simulink model "hw_CS1A_seq"  (R2025b)
settings: Solver=FixedStepAuto  StartTime=0.0  StopTime=inf  RelTol=1e-3  EnableMultiTasking=on
InitFcn:
  | run(fullfile(fileparts(get_param(bdroot,'FileName')),'Hardware_settings.m'));
  | run(fullfile(fileparts(get_param(bdroot,'FileName')),'ref_sequence_settings.m'));
StopFcn:
  | run(fullfile(fileparts(get_param(bdroot,'FileName')),'Hardware_data_save.m'));
values from neighbouring files (symbols this model uses):
  ref_hold_s = 8    [ref_sequence_settings.m]
  ref_seq_deg = [45 -45 90 0 -90 0]    [ref_sequence_settings.m]
  ts = 1/1000    (= 0.001)    [Hardware_settings.m]    (also in data_test_06.mat; qube_model.m)
libraries: simulink_extras x4, simulink x3, arduinolib x1
settings Model: SimulationMode=external  ExtModeTrigDuration=2  Creator=ricardoaguilera  LastModifiedBy=jaylen
settings SolverCC: AutoInsertRateTranBlk=on
settings DataIOCC: ReturnWorkspaceOutputs=off
settings OptimizationCC: EnhancedBackFolding=on  PassReuseOutputArgsAs=Individual arguments  ZeroExternalMemoryAtStartup=off  ZeroInternalMemoryAtStartup=off  MaxStackSize=64  OptimizeBlockOrder=speed  DifferentSizesBufferReuse=on  OptimizationCustomize=off  EfficientTunableParamExpr=on
settings DebuggingCC: ParameterTunabilityLossMsg=error
settings HardwareCC: ProdBitPerPointer=32.0  ProdBitPerSizeT=32.0  ProdBitPerPtrDiffT=32.0  ProdLargestAtomicInteger=Long  ProdLargestAtomicFloat=Double  ProdWordSize=32.0  ProdHWDeviceType=ARM Compatible->ARM Cortex
settings SFSimCC: MATLABDynamicMemAlloc=off
settings RTWCC: SystemTargetFile=ert.tlc  HardwareBoard=Teensy 4.1 (Arduino Compatible)  TemplateMakefile=ert_default_tmf  Toolchain=Arduino ARM M7  BuildConfiguration=Faster Runs  Description=Embedded Coder
settings CodeAppCC: ForceParamTrailComments=on  IgnoreCustomStorageClasses=off  OperatorAnnotations=on  SimulinkDataObjDesc=on  SFDataObjDesc=on  InsertBlockDesc=on
settings ERTTargetCC: ExtModeTransport=3.0  ExtModeStaticAlloc=on  ExtModeAutomaticAllocSize=off  ExtModeStaticAllocSize=65536.0  ExtModeMexFile=ext_xcp  ExtModeIntrfLevel=Level2 - Open  InlinedParameterPlacement=Hierarchical  SupportContinuousTime=on  SupportVariableSizeSignals=on

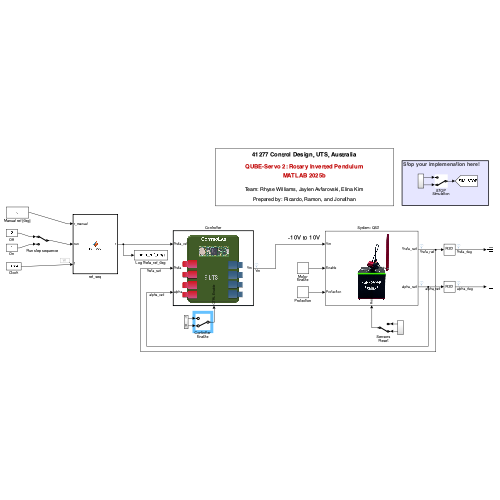
[thumbnail: Simulink's stored preview of the top-level diagram]
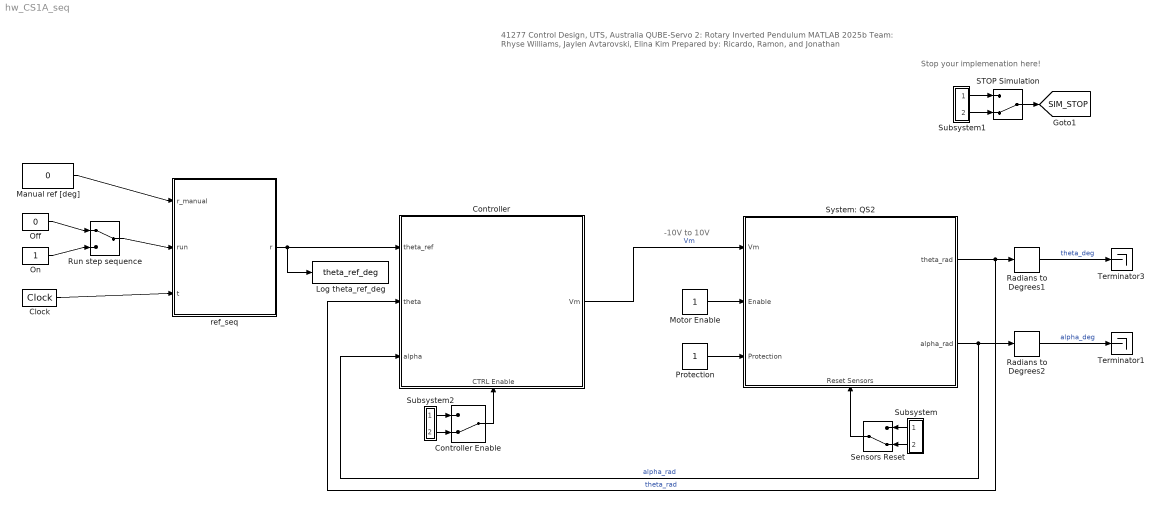
== system hw_CS1A_seq ==
  note: Stop your implemenation here!
  note: -10V to 10V
  note: 41277 Control Design, UTS, Australia
      |
      | QUBE-Servo 2: Rotary Inverted Pendulum
      |
      | MATLAB 2025b
      |
      | Team: Rhyse Williams, Jaylen Avtarovski, Elina Kim
      |
      | Prepared by: Ricardo, Ramon, and Jonathan
  Clock : DigitalClock  SampleTime=ts
  Controller : Subsystem  TreatAsAtomicUnit=on
      settings: PortSchema="{\"entries\":[{\"content\":{\"sides\":[{\"content\":{\"connectorIds\":[\"In1\",\"In2\",\"In3\"]},\"type\":\"ConnectorPlacement.EquallySpacedRectSide\",\"uuid\":\"0746f990-c749-44b4-b231-71e9c63a70c9\"},{\"content\":{\"connectorIds\":[\"Out1\"],\"side\":\"RIGHT\"},\"type\":\"ConnectorPlacement.EquallySpacedRectSide\",\"uuid\":\"2be26398-fce4-47ae-bcef-dcf9a7bb9bcb\"},{\"content\":{\"side\":\"TOP\"},\"type\":\"ConnectorPlacement.EquallySpacedRectSide\",\"uuid\":\"03fd616b-3dd6-472f-b1cd-bcbe330f410d\"},{\"content\":{\"connectorIds\":[\"In4\"],\"side\":\"BOTTOM\"},\"type\":\"ConnectorPlacement.EquallySpacedRectSide\",\"uuid\":\"e0197938-1dca-4730-aea1-41c64defbdb5\"}]},\"type\":\"ConnectorPlacement.EquallySpacedConnector\",\"uuid\":\"8db17840-dba9-44ab-b10b-ffa616c53e04\"}],\"packageUris\":[\"http://schema.mathworks.com/mf0/Connector/R2020b\"],\"version\":\"1.0\"}"
      mask Display: image('Board.png');
  Controller Enable : ManualSwitch  CurrentSetting=0
  Log theta_ref_deg : ToWorkspace  VariableName=theta_ref_deg  SampleTime=-1
  Manual ref [deg] : Constant  Value=0
  Motor Enable : Constant
  Off : Constant  Value=0
  On : Constant
  Protection : Constant
  Radians to Degrees1 : simulink_extras/Transformations/Radians to Degrees
  Radians to Degrees2 : simulink_extras/Transformations/Radians to Degrees
  Run step sequence : ManualSwitch
  STOP Simulation : ManualSwitch  CurrentSetting=0
  Sensors Reset : ManualSwitch  CurrentSetting=0
  Subsystem : Subsystem
  Subsystem1 : Subsystem
  Subsystem2 : Subsystem
  "System: QS2      " : Subsystem
      settings: PortSchema="{\"entries\":[{\"content\":{\"sides\":[{\"content\":{\"connectorIds\":[\"In1\",\"In2\",\"In3\"]},\"type\":\"ConnectorPlacement.EquallySpacedRectSide\",\"uuid\":\"0610958f-a0ee-4862-9bf4-da2decae3359\"},{\"content\":{\"connectorIds\":[\"Out1\",\"Out2\"],\"side\":\"RIGHT\"},\"type\":\"ConnectorPlacement.EquallySpacedRectSide\",\"uuid\":\"1dc03bce-2cf3-4202-8885-89b5465dfc9c\"},{\"content\":{\"side\":\"TOP\"},\"type\":\"ConnectorPlacement.EquallySpacedRectSide\",\"uuid\":\"bdedebb1-69f1-406e-86fb-8ca91daed26d\"},{\"content\":{\"connectorIds\":[\"In4\"],\"side\":\"BOTTOM\"},\"type\":\"ConnectorPlacement.EquallySpacedRectSide\",\"uuid\":\"304d8cf9-f7c8-4566-8aa8-5eccf9f2ddf3\"}]},\"type\":\"ConnectorPlacement.EquallySpacedConnector\",\"uuid\":\"5c4cc706-3b46-49e2-ad64-d3400bef9abc\"}],\"packageUris\":[\"http://schema.mathworks.com/mf0/Connector/R2020b\"],\"version\":\"1.0\"}"
      mask Display: image('QUBE-Servo3-front-1.png', [10,0,10,0,100,100]);
  Terminator1 : Terminator
  Terminator3 : Terminator
  ref_seq : MATLAB Function  TreatAsAtomicUnit=on
  tag scope: SIM_STOP=global
  wires:
  Motor Enable/1 -> "System: QS2      "/2(Enable)
  Controller/1(Vm) -> "System: QS2      "/1(Vm)  "Vm"
  "System: QS2      "/2(alpha_rad) -> Radians to Degrees2/1, Controller/3(alpha)  "alpha_rad"
  "System: QS2      "/1(theta_rad) -> Radians to Degrees1/1, Controller/2(theta)  "theta_rad"
  Protection/1 -> "System: QS2      "/3(Protection)
  Radians to Degrees1/1 -> Terminator3/1  "theta_deg"
  Radians to Degrees2/1 -> Terminator1/1  "alpha_deg"
  Subsystem/1(" ") -> Sensors Reset/1
  Subsystem/2("  ") -> Sensors Reset/2
  Sensors Reset/1 -> "System: QS2      "/4(Reset Sensors)
  Subsystem1/1(" ") -> STOP Simulation/1
  Subsystem1/2("  ") -> STOP Simulation/2
  STOP Simulation/1 -> [SIM_STOP]
  Subsystem2/1(1) -> Controller Enable/1
  Subsystem2/2(0) -> Controller Enable/2
  Controller Enable/1 -> Controller/4(CTRL Enable)
  ref_seq/1(r) -> Controller/1(theta_ref), Log theta_ref_deg/1
  Clock/1 -> ref_seq/3(t)
  Run step sequence/1 -> ref_seq/2(run)
  Off/1 -> Run step sequence/1
  Manual ref [deg]/1 -> ref_seq/1(r_manual)
  On/1 -> Run step sequence/2

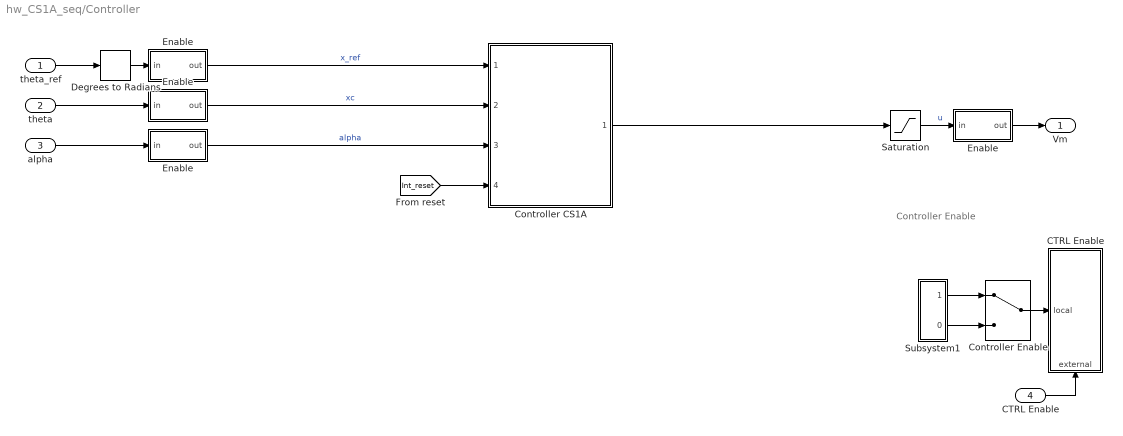
== system hw_CS1A_seq/Controller ==
  note: Controller Enable
  theta_ref : Inport
  theta : Inport  Port=2
  alpha : Inport  Port=3
  CTRL Enable : Inport  Port=4
  "  Enable" : Subsystem
  " Enable" : Subsystem
  "CTRL Enable " : Subsystem
      settings: PortSchema="{\"entries\":[{\"content\":{\"sides\":[{\"content\":{\"connectorIds\":[\"In1\"]},\"type\":\"ConnectorPlacement.EquallySpacedRectSide\",\"uuid\":\"17c10e5b-e4eb-4ba8-8e00-f6bd1827336e\"},{\"content\":{\"side\":\"RIGHT\"},\"type\":\"ConnectorPlacement.EquallySpacedRectSide\",\"uuid\":\"28de4c7e-9722-4e76-ae90-e2752cb22a9a\"},{\"content\":{\"side\":\"TOP\"},\"type\":\"ConnectorPlacement.EquallySpacedRectSide\",\"uuid\":\"1d73f9a3-eba4-4b67-a490-c6a9248242c0\"},{\"content\":{\"connectorIds\":[\"In2\"],\"side\":\"BOTTOM\"},\"type\":\"ConnectorPlacement.EquallySpacedRectSide\",\"uuid\":\"c2b41749-95c8-42da-9d5d-86e4b8e938ea\"}]},\"type\":\"ConnectorPlacement.EquallySpacedConnector\",\"uuid\":\"ba6dba79-b206-47dc-8f48-5bdedca08d9e\"}],\"packageUris\":[\"http://schema.mathworks.com/mf0/Connector/R2020b\"],\"version\":\"1.0\"}"
  Controller Enable : ManualSwitch
  Controller CS1A : Subsystem  ReferencedSubsystem=ctrl_CS1A
  Degrees to Radians : simulink_extras/Transformations/Degrees to Radians
  Enable : Subsystem
  "Enable " : Subsystem
  Saturation : Saturate  UpperLimit=10  LowerLimit=-10
  Subsystem1 : Subsystem
  Vm : Outport
  wires:
  theta_ref/1 -> Degrees to Radians/1
  Subsystem1/2(0) -> Controller Enable/2
  Subsystem1/1(1) -> Controller Enable/1
  CTRL Enable/1 -> "CTRL Enable "/2(external)
  Controller Enable/1 -> "CTRL Enable "/1(local)
  Degrees to Radians/1 -> "  Enable"/1(in)
  theta/1 -> "Enable "/1(in)
  alpha/1 -> " Enable"/1(in)
  Enable/1(out) -> Vm/1
  Saturation/1 -> Enable/1(in)  "u"
  "  Enable"/1(out) -> Controller CS1A/1  "x_ref"
  "Enable "/1(out) -> Controller CS1A/2  "xc"
  " Enable"/1(out) -> Controller CS1A/3  "alpha"
  [Int_reset] -> Controller CS1A/4
  Controller CS1A/1 -> Saturation/1

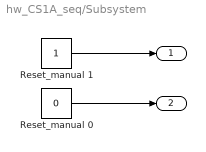
== system hw_CS1A_seq/Subsystem ==
  Reset_manual 0 : Constant  Value=0  SampleTime=-1
  Reset_manual 1 : Constant  SampleTime=-1
  " " : Outport
  "  " : Outport  Port=2
  wires:
  Reset_manual 1/1 -> " "/1
  Reset_manual 0/1 -> "  "/1

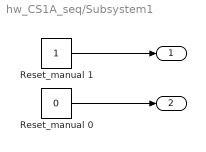
== system hw_CS1A_seq/Subsystem1 ==
  Reset_manual 0 : Constant  Value=0  SampleTime=-1
  Reset_manual 1 : Constant  SampleTime=-1
  " " : Outport
  "  " : Outport  Port=2
  wires:
  Reset_manual 1/1 -> " "/1
  Reset_manual 0/1 -> "  "/1

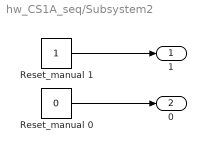
== system hw_CS1A_seq/Subsystem2 ==
  Reset_manual 0 : Constant  Value=0  SampleTime=-1
  Reset_manual 1 : Constant  SampleTime=-1
  1 : Outport
  0 : Outport  Port=2
  wires:
  Reset_manual 1/1 -> 1/1
  Reset_manual 0/1 -> 0/1

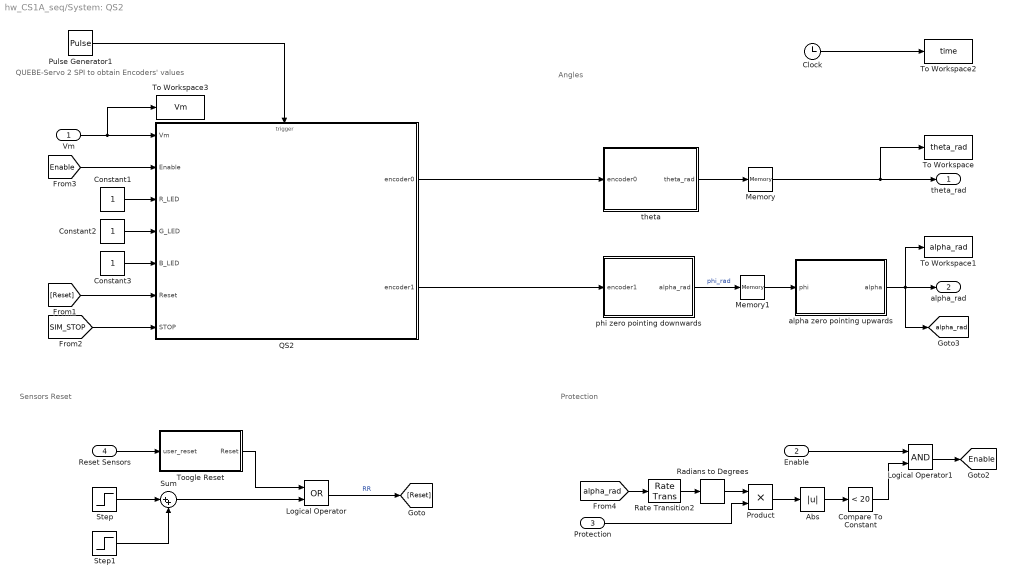
== system hw_CS1A_seq/System: QS2       ==
  note: QUEBE-Servo 2 SPI to obtain Encoders' values
  note: Sensors Reset
  note: Protection
  note: Angles
  Vm : Inport
  Enable : Inport  Port=2
  Protection : Inport  Port=3
  Reset Sensors : Inport  Port=4
  Abs : Abs  SaturateOnIntegerOverflow=off
  Clock : Clock
  Compare To Constant : simulink/Logic and Bit Operations/Compare To Constant  relop=<  const=20  OutDataTypeStr=boolean
  Constant1 : Constant
  Constant2 : Constant
  Constant3 : Constant
  Logical Operator : Logic  Operator=OR  AllPortsSameDT=off  OutDataTypeStr=boolean
  Logical Operator1 : Logic  AllPortsSameDT=off  OutDataTypeStr=boolean
  Memory : Memory
  Memory1 : Memory
  Product : Product
  Pulse Generator1 : DiscretePulseGenerator  PulseType=Time based  Period=ts  PulseWidth=50
  QS2 : Subsystem  TreatAsAtomicUnit=on
      mask Display: image('SPI.png');
  Radians to Degrees : simulink_extras/Transformations/Radians to Degrees
  Rate Transition2 : RateTransition  OutPortSampleTimeOpt=Inherit  OutPortSampleTimeMultiple=2
  Step : Step  Time=ts
  Step1 : Step  Time=2*ts  After=-1
  Sum : Sum  Inputs=|++
  To Workspace : ToWorkspace  VariableName=theta_rad  SampleTime=-1
  To Workspace1 : ToWorkspace  VariableName=alpha_rad  SampleTime=-1
  To Workspace2 : ToWorkspace  VariableName=time  SampleTime=-1
  To Workspace3 : ToWorkspace  VariableName=Vm  SampleTime=-1
  Toogle Reset : MATLAB Function  TreatAsAtomicUnit=on  SystemSampleTime=ts
  alpha zero pointing upwards : MATLAB Function  TreatAsAtomicUnit=on
  phi zero pointing downwards : MATLAB Function  TreatAsAtomicUnit=on
  theta : MATLAB Function  TreatAsAtomicUnit=on
  theta_rad : Outport
  alpha_rad : Outport  Port=2
  tag scope: Enable=global, alpha_rad=global
  wires:
  Toogle Reset/1(Reset) -> Logical Operator/1
  Logical Operator/1 -> [Reset]  "RR"
  Step/1 -> Sum/1
  Step1/1 -> Sum/2
  Sum/1 -> Logical Operator/2
  Pulse Generator1/1 -> QS2/Trigger
  [Reset] -> QS2/6(Reset)
  Vm/1 -> To Workspace3/1, QS2/1(Vm)
  theta/1(theta_rad) -> Memory/1
  phi zero pointing downwards/1(alpha_rad) -> Memory1/1  "phi_rad"
  Abs/1 -> Compare To Constant/1
  [Enable] -> QS2/2(Enable)
  QS2/1(encoder0) -> theta/1(encoder0)
  Rate Transition2/1 -> Radians to Degrees/1
  Logical Operator1/1 -> [Enable]
  Compare To Constant/1 -> Logical Operator1/2
  Enable/1 -> Logical Operator1/1
  Protection/1 -> Product/2
  QS2/2(encoder1) -> phi zero pointing downwards/1(encoder1)
  Product/1 -> Abs/1
  [alpha_rad] -> Rate Transition2/1
  Radians to Degrees/1 -> Product/1
  Memory/1 -> To Workspace/1, theta_rad/1
  Memory1/1 -> alpha zero pointing upwards/1(phi)
  alpha zero pointing upwards/1(alpha) -> To Workspace1/1, alpha_rad/1, [alpha_rad]
  Constant1/1 -> QS2/3(R_LED)
  Constant2/1 -> QS2/4(G_LED)
  Constant3/1 -> QS2/5(B_LED)
  Reset Sensors/1 -> Toogle Reset/1(user_reset)
  [SIM_STOP] -> QS2/7(STOP)
  Clock/1 -> To Workspace2/1

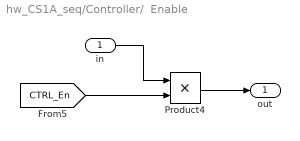
== system hw_CS1A_seq/Controller/  Enable ==
  in : Inport
  Product4 : Product
  out : Outport
  wires:
  in/1 -> Product4/1
  Product4/1 -> out/1
  [CTRL_En] -> Product4/2

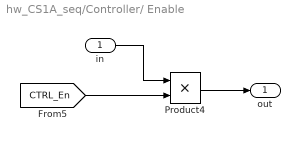
== system hw_CS1A_seq/Controller/ Enable ==
  in : Inport
  Product4 : Product
  out : Outport
  wires:
  in/1 -> Product4/1
  Product4/1 -> out/1
  [CTRL_En] -> Product4/2

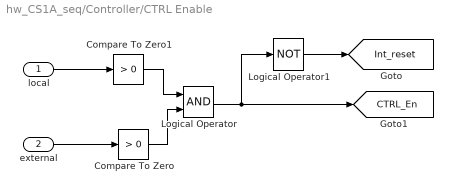
== system hw_CS1A_seq/Controller/CTRL Enable  ==
  local : Inport
  external : Inport  Port=2
  Compare To Zero : simulink/Logic and Bit Operations/Compare To Zero  relop=>  OutDataTypeStr=boolean
  Compare To Zero1 : simulink/Logic and Bit Operations/Compare To Zero  relop=>  OutDataTypeStr=boolean
  Logical Operator : Logic  AllPortsSameDT=off  OutDataTypeStr=boolean
  Logical Operator1 : Logic  Operator=NOT  AllPortsSameDT=off  OutDataTypeStr=boolean
  tag scope: CTRL_En=global, Int_reset=global
  wires:
  Logical Operator/1 -> [CTRL_En], Logical Operator1/1
  external/1 -> Compare To Zero/1
  local/1 -> Compare To Zero1/1
  Compare To Zero1/1 -> Logical Operator/1
  Compare To Zero/1 -> Logical Operator/2
  Logical Operator1/1 -> [Int_reset]

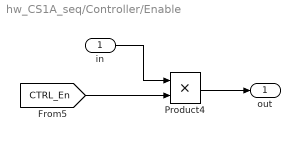
== system hw_CS1A_seq/Controller/Enable ==
  in : Inport
  Product4 : Product
  out : Outport
  wires:
  in/1 -> Product4/1
  Product4/1 -> out/1
  [CTRL_En] -> Product4/2

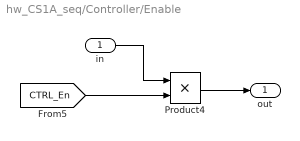
== system hw_CS1A_seq/Controller/Enable  ==
  in : Inport
  Product4 : Product
  out : Outport
  wires:
  [CTRL_En] -> Product4/2
  Product4/1 -> out/1
  in/1 -> Product4/1

== system hw_CS1A_seq/Controller/Subsystem1 ==
  Reset_manual 0 : Constant  Value=0  SampleTime=-1
  Reset_manual 1 : Constant  SampleTime=-1
  1 : Outport
  0 : Outport  Port=2
  wires:
  Reset_manual 1/1 -> 1/1
  Reset_manual 0/1 -> 0/1

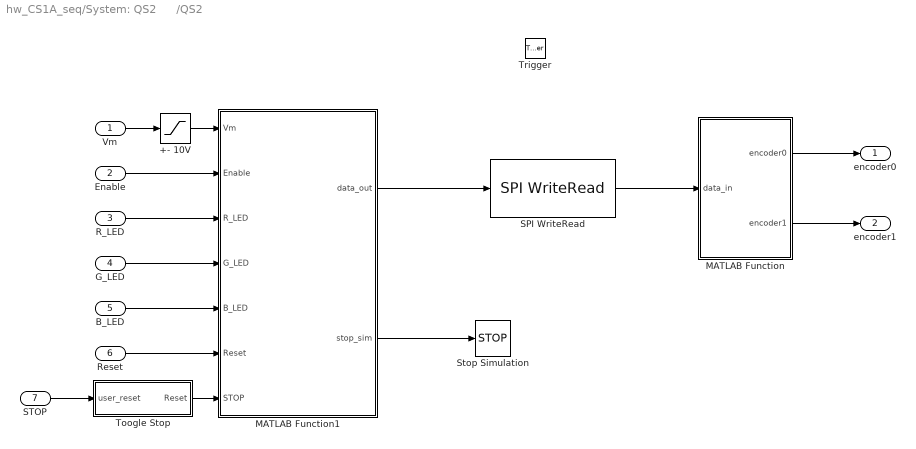
== system hw_CS1A_seq/System: QS2      /QS2 ==
  Vm : Inport
  Enable : Inport  Port=2
  R_LED : Inport  Port=3
  G_LED : Inport  Port=4
  B_LED : Inport  Port=5
  Reset : Inport  Port=6
  STOP : Inport  Port=7
  Trigger : TriggerPort  VariantControl=(inherit)
  +- 10V : Saturate  UpperLimit=10  LowerLimit=-10
  MATLAB Function : MATLAB Function  TreatAsAtomicUnit=on
  MATLAB Function1 : MATLAB Function  TreatAsAtomicUnit=on
  SPI WriteRead : arduinolib/SPI WriteRead  SPIModule=0  slaveSelectPin_=10  blockPlatform=ARDUINO
  Stop Simulation : Stop
  Toogle Stop : MATLAB Function  TreatAsAtomicUnit=on
  encoder0 : Outport
  encoder1 : Outport  Port=2
  wires:
  Enable/1 -> MATLAB Function1/2(Enable)
  G_LED/1 -> MATLAB Function1/4(G_LED)
  MATLAB Function1/1(data_out) -> SPI WriteRead/1
  Vm/1 -> +- 10V/1
  R_LED/1 -> MATLAB Function1/3(R_LED)
  B_LED/1 -> MATLAB Function1/5(B_LED)
  Reset/1 -> MATLAB Function1/6(Reset)
  +- 10V/1 -> MATLAB Function1/1(Vm)
  STOP/1 -> Toogle Stop/1(user_reset)
  MATLAB Function1/2(stop_sim) -> Stop Simulation/1
  SPI WriteRead/1 -> MATLAB Function/1(data_in)
  MATLAB Function/1(encoder0) -> encoder0/1
  MATLAB Function/2(encoder1) -> encoder1/1
  Toogle Stop/1(Reset) -> MATLAB Function1/7(STOP)

== matlab function hw_CS1A_seq/System: QS2      /QS2/MATLAB Function1 ==
  data: Vm input; Enable input; R_LED input; data_out output size=17; G_LED input; B_LED input; Reset input; STOP input; stop_sim output size=1
function [data_out,stop_sim]  = QS2_SPI_write(Vm,Enable,R_LED,G_LED,B_LED,Reset, STOP)

persistent count_startup count_stop stop
if isempty(count_startup)
    count_startup = 1; 
    count_stop = 1;
    stop = false;
end

if (STOP > 0)
    stop = true;
end

startup = true;
if (count_startup>=5)
    startup = false;
    count_startup = 10;
end

%% SPI data to be sent
SPI_data_out = uint8(zeros(17,1));
SPI_data_out(1) = 1;
writeMask = 31;
SPI_data_out(3) = writeMask;

%% Motor Voltage
Vm_int = int16(Vm *(625.0 / 15.0));
Vm_int = bitset(Vm_int,16);
motor = typecast(Vm_int,'uint16');
motorMSB = bitshift(motor,-8);
motorLSB = bitand(motor,255);

SPI_data_out(16) = motorMSB;
SPI_data_out(17) = motorLSB;


%% Enable
if (Enable~=1)
    writeMask = 31;
    SPI_data_out(3) = writeMask;
    SPI_data_out(16) = 0;
    SPI_data_out(17) = 0;
    %R_LED = 1;
    %G_LED = 0;
    %B_LED = 0;
end

%% Reset Encoders
if (Reset || startup)
    writeMask = 127;
    SPI_data_out(3) = writeMask;
    SPI_data_out(16) = 0;
    SPI_data_out(17) = 0;
    %R_LED = 1;
    %G_LED = 1;
    %B_LED = 1;
end

stop_sim = false;
if (stop || count_stop>1)
    count_stop = count_stop + 1;
    writeMask = 31;
    SPI_data_out(3) = writeMask;
    SPI_data_out(16) = 0;
    SPI_data_out(17) = 0;
    %R_LED = 1;
    %G_LED = 0;
    %B_LED = 0;
end

if (count_stop> 1)
    stop_sim = true;
end

count_startup = count_startup + 1;


%% LEDs
R_LED = 999*min(1, max(0, R_LED));
G_LED = 999*min(1, max(0, G_LED));
B_LED = 999*min(1, max(0, B_LED));

LEDRedMSB   = bitshift(R_LED,-8);
LEDRedLSB   = bitand(R_LED, 255);
LEDGreenMSB = bitshift(G_LED,-8);
LEDGreenLSB = bitand(G_LED, 255);
LEDBlueMSB  = bitshift(B_LED,-8);
LEDBlueLSB  = bitand(B_LED, 255);


SPI_data_out(4) = LEDRedMSB;
SPI_data_out(5) = LEDRedLSB;
SPI_data_out(6) = LEDGreenMSB;
SPI_data_out(7) = LEDGreenLSB;
SPI_data_out(8) = LEDBlueMSB;
SPI_data_out(9) = LEDBlueLSB;

data_out = SPI_data_out;

== matlab function hw_CS1A_seq/System: QS2      /phi zero pointing downwards ==
  data: encoder1 input size=1; alpha_rad output size=1
function alpha_rad = enc2alpha(encoder1)
%calibrate this angle sensor


% encoder provides 2048 counts per rotation
% when encoder1 = 0 --> alpha = -pi

% Convert E1 counts to pendulum angle (radians)
alpha_rad = encoder1 * (2*pi/2048);

== matlab function hw_CS1A_seq/System: QS2      /theta ==
  data: encoder0 input size=1; theta_rad output size=1
function theta_rad = enc2theta(encoder0)
%calibrate this angle sensor

% encoder provides 2048 counts per rotation
% when encoder0 = 0 --> alpha = 0
% negative rotation
theta_rad = encoder0 * (2*pi/2048);
% Convert E0 counts to rotation angle (radians)
%theta_rad =encoder0;

== matlab function hw_CS1A_seq/System: QS2      /alpha zero pointing upwards ==
  data: phi input; alpha output
function alpha = fcn(phi)

phi = wrapTo2Pi(phi); % keep phi \in [0, 2*pi]

alpha = phi - pi; % alpha \in [-pi, pi]

== matlab function hw_CS1A_seq/System: QS2      /QS2/MATLAB Function ==
  data: data_in input size=17; encoder0 output size=1; encoder1 output size=1
function [encoder0, encoder1] =  QS2_SPI_read(data_in)

%% Encoder 0

%encoder0 data
encoder0Byte = [data_in(5), data_in(4), data_in(3)];

% Build 24-bit value
enc24 = bitor( ...
          bitor(bitshift(uint32(encoder0Byte(3)),16), ...
                bitshift(uint32(encoder0Byte(2)),8)), ...
          uint32(encoder0Byte(1)));

% Sign-extend 24-bit to 32-bit:
% left shift 8, then arithmetic right shift 8 (on int32) 
enc0 = bitshift(bitshift(int32(enc24), 8), -8);
encoder0 = double(enc0);

%% Encoder 1

%encoder1 data
encoder1Byte = [data_in(8), data_in(7), data_in(6)];

% Build 24-bit unsigned value
enc24 = bitor( ...
          bitor(bitshift(uint32(encoder1Byte(3)),16), ...
                bitshift(uint32(encoder1Byte(2)),8)), ...
          uint32(encoder1Byte(1)));

% Sign-extend from 24-bit to int32
enc1 = bitshift(bitshift(int32(enc24), 8), -8);

% Wrap counts to [0, 2047]
enc1 = mod(enc1, 2048);
if enc1 < 0
    enc1 = enc1 + 2048;
end
encoder1 = double(enc1);

== matlab function hw_CS1A_seq/ref_seq ==
  data: r_manual input; r output; run input; t input; ref_seq_deg parameter; ref_hold_s parameter
function r = ref_seq(r_manual, run, t, ref_seq_deg, ref_hold_s)
%REF_SEQ Timed arm step sequence, started by the "Run step sequence" switch.
persistent t0 active
if isempty(t0)
    t0 = 0;
    active = false;
end
if run > 0.5
    if ~active                 % switch just turned on: restart the sequence
        t0 = t;
        active = true;
    end
    k = floor((t - t0)/ref_hold_s) + 1;
    k = min(max(k, 1), numel(ref_seq_deg));
    r = ref_seq_deg(k);
else
    active = false;
    r = r_manual;
end

== matlab function hw_CS1A_seq/System: QS2      /QS2/Toogle Stop ==
  data: Reset output; user_reset input
function Reset = fcn(user_reset)

persistent reset_in_prev count

if isempty(reset_in_prev)
    reset_in_prev = false;
    count = 1;
end

reset_in = false;
if (user_reset>0.5)
    reset_in = true;
end


% Detect the moment the manual switch is flipped
Reset = 0;
if(reset_in ~= reset_in_prev && count > 5)
    Reset = 1; 
end
reset_in_prev = reset_in;
count = count + 1;
if (count >5)
    count = 10;
end

end

== matlab function hw_CS1A_seq/System: QS2      /Toogle Reset ==
  data: Reset output; user_reset input
function Reset = fcn(user_reset)

persistent reset_in_prev

if isempty(reset_in_prev)
    reset_in_prev = false;
end

reset_in = false;
if (user_reset>0.5)
    reset_in = true;
end


% Detect the moment the manual switch is flipped
Reset = 0;
if(reset_in ~= reset_in_prev)
    Reset = 1; 
end
reset_in_prev = reset_in;

end
